simulink model "Prey_Predator_STM32F4"  (R2025a)
settings: Solver=FixedStepDiscrete  StartTime=0.0  StopTime=10.0  RelTol=1e-3
PreLoadFcn:
  | waijung.modelPreload; % Required for working with Waijung Blockset. Do not remove.
undefined symbols (not defined in the file): HSEOSC, Link, LQFP176, ST, STM32F417IG
libraries: stm32f4_io_lib x144, fuzblock x1, stm32f4_device_config_lib x1
(part 1 of 3)
CloseFcn:
  | waijung.modelClose; % Required for working with Waijung Blockset. Do not remove.
settings Model: Creator=Krisada  LastModifiedBy=prizy
settings SolverCC: AlgebraicLoopSolver=TrustRegion
settings DataIOCC: LimitDataPoints=on  SaveFormat=Array  SignalLoggingSaveFormat=ModelDataLogs  ReturnWorkspaceOutputs=off
settings OptimizationCC: ExpressionDepthLimit=2147483647.0  LifeSpan=1  EfficientTunableParamExpr=on
settings DebuggingCC: UnderspecifiedInitializationDetection=Classic  MergeDetectMultiDrivingBlocksExec=none  SolverPrmCheckMsg=warning  ParameterPrecisionLossMsg=none  FcnCallInpInsideContextMsg=warning  UnconnectedInputMsg=warning  UnconnectedOutputMsg=warning  UnconnectedLineMsg=warning  StateNameClashWarn=warning  SFUnexpectedBacktrackingDiag=warning  SFNoUnconditionalDefaultTransitionDiag=warning  SFExecutionAtInitializationDiag=none  ArithmeticOperatorsInVariantConditions=warning
settings HardwareCC: ProdBitPerPointer=32.0  ProdBitPerSizeT=32.0  ProdBitPerPtrDiffT=32.0  ProdLargestAtomicFloat=None  ProdIntDivRoundTo=Undefined  ProdWordSize=32.0  ProdHWDeviceType=ARM Compatible->Cortex - M4  TargetEndianess=LittleEndian  TargetHWDeviceType=ARM Compatible->Cortex - M4
settings ModelReferenceCC: PropagateSignalLabelsOutOfModel=off
settings SFSimCC: SimUseLocalCustomCode=off  MATLABDynamicMemAlloc=off  CustomCodeUndefinedFunction=UseInterfaceOnly
settings RTWCC: SystemTargetFile=stm32f4.tlc  GenerateMakefile=off  TemplateMakefile=ert_default_tmf  RTWUseLocalCustomCode=off  GPUComputeCapability=3.5  Description=STM32F4 Target
settings CodeAppCC: IgnoreCustomStorageClasses=off  CustomSymbolStrType=$N$R$M  StateflowObjectComments=on  InternalIdentifier=Classic
settings STFCustomTargetCC: SystemTargetFile=stm32f4.tlc  MultiwordLength=2048.0  DynamicStringBufferSize=256.0  ModelReferenceCompliant=off  CombineOutputUpdateFcns=on  ERTCustomFileBanners=on  SupportContinuousTime=off  SupportNonInlinedSFcns=off  RemoveResetFunc=on  MATLABClassNameForMDSCustomization=Simulink.SoftwareTarget.ERTCustomization  GRTInterface=off
settings ERTTargetCC: ExtModeTransport=0.0  ExtModeStaticAlloc=off  ExtModeMexFile=noextcomm  ExtModeIntrfLevel=Level1  InlinedParameterPlacement=Hierarchical  ERTSrcFileBannerTemplate=stm32f4_code_template.cgt  ERTHdrFileBannerTemplate=stm32f4_code_template.cgt  ERTDataSrcFileTemplate=stm32f4_code_template.cgt  ERTDataHdrFileTemplate=stm32f4_code_template.cgt  ERTCustomFileTemplate=stm32f4_file_process.tlc  ConvertIfToSwitch=off  SuppressUnreachableDefaultCases=off  DynamicArrayContainerType=coder::array  MultiwordLength=2048.0  ModelReferenceCompliant=off  ParMdlRefBuildCompliant=off  CompOptLevelCompliant=off  ConcurrentExecutionCompliant=off  ModelStepFunctionPrototypeControlCompliant=off  CPPClassGenCompliant=off  UseToolchainInfoCompliant=off
settings ConfigComp: CovMetricSettings=dw  CovSaveCumulativeToWorkspaceVar=on  CovSaveSingleToWorkspaceVar=on  CovExternalEMLEnable=off

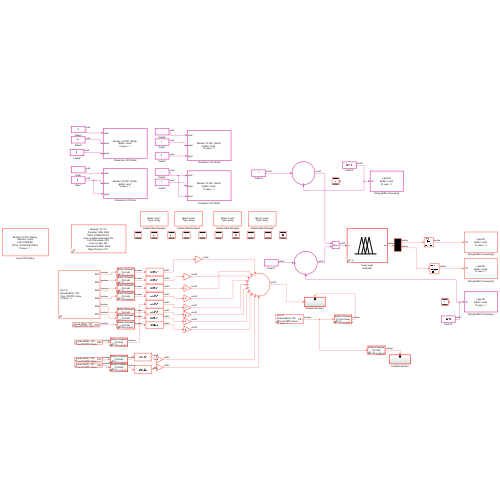
[thumbnail: Simulink's stored preview of the top-level diagram]
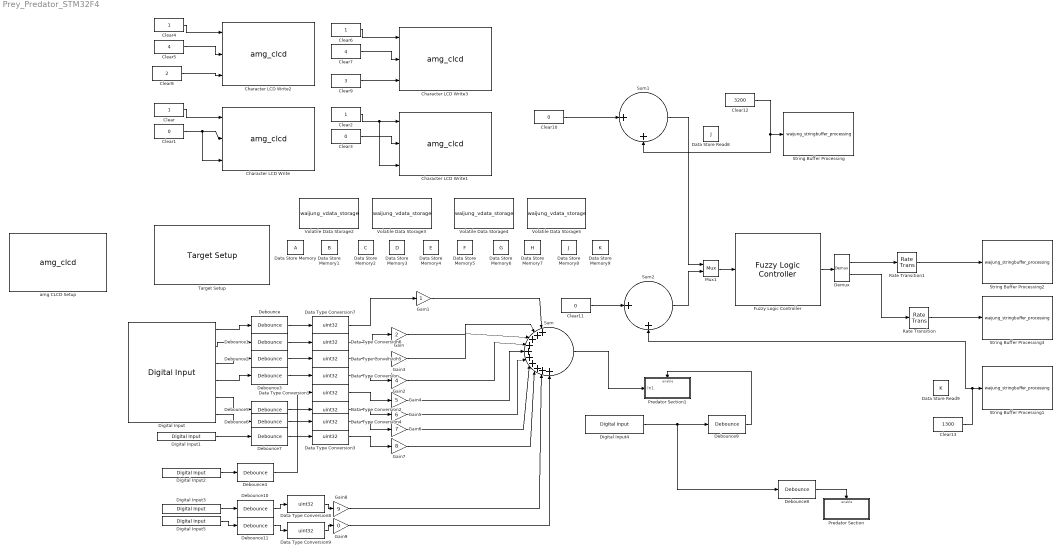
== system Prey_Predator_STM32F4 ==
  Character LCD Write : S-Function  FunctionName=amg_clcd  Parameters=module,configuration,inputtypearray,outputtypearray,confstr,sampletime,sampletimestr,blockid  SFunctionDeploymentMode=off  EnableBusSupport=off  mask(amg_clcd){configuration=Transaction, module=1, model=amg CLCD Std, interface=4-bits, linecount=4, columncount=20, gpiotype=Push-pull, controlport=E, control_rs=15, control_rw=13, control_en=11, dataport=A, data0=7, data1=5, data2=3, data3=1, usestringbuffer=on, stringbuffer=Line1, varname=VolatileDataStorage2_Line1, inputtypearray=[3 -1 -1 -1], outputtypearray=[0], confstr=["4","4","20","PP","E","15","11","13","","A","","","","","7","5","3","1","1","VolatileDataStorage2_Line1","1","0","0","0","1","0","0","0","0","stm32f4"], sampletime=-1, sampletimestr=-1, blockid=CharacterLCDWrite}
      mask prompts: model "LCD model:"; linecount "Number of lines:"; columncount "Number of columns:"; gpiotype "GPIO Output type:"; controlport "GPIO control port:"; control_rs "GPIO control pin, RS:"; control_rw "GPIO control pin, RW:"; control_en "GPIO control pin, EN:"; dataport "GPIO data D[7:4] port"; data0 "GPIO data pin, D4:"; data1 "GPIO data pin, D5:"; data2 "GPIO data pin, D6:"; data3 "GPIO data pin, D7:"; usestringbuffer "Use string buffer"; stringbuffer "String buffer"; varname "Variable name"; inputtypearray "Input type array"; outputtypearray "Output type array"; confstr "Configuration string"; sampletime "Sample time (sec)"; sampletimestr "Compiled sample time (sec) in string"
      mask help:
      | Note for cmd:
      | 1 - Clear specified LCD line display before write data to LCD.
      | Otherwise (e.g. 0) - Write data without clearing LCD Line.
      |
      | Position:
      | x = 0, First Character (from left to right)
      | y = 0, Top Line
      mask init:
      | amg_clcd_callback('init');
      mask Help: web(fullfile(waijungdocroot,'amg_clcd_write.htm'), '-browser')
      mask TypeOptions configuration: Setup | Transaction
      mask Callback configuration: amg_clcd_callback('configuration');
      mask TypeOptions module: 1 | 2 | 3 | 4
      mask TypeOptions model: amg CLCD Std
      mask TypeOptions interface: 4-bits
      mask TypeOptions gpiotype: Push-pull | Open-drain
      mask TypeOptions controlport: A | B | C | D | E | F | G | H | I
      mask TypeOptions control_rs: 0 | 1 | 2 | 3 | 4 | 5 | 6 | 7 | 8 | 9 | 10 | 11 | 12 | 13 | 14 | 15
      mask TypeOptions control_rw: 0 | 1 | 2 | 3 | 4 | 5 | 6 | 7 | 8 | 9 | 10 | 11 | 12 | 13 | 14 | 15
      mask TypeOptions control_en: 0 | 1 | 2 | 3 | 4 | 5 | 6 | 7 | 8 | 9 | 10 | 11 | 12 | 13 | 14 | 15
      mask TypeOptions dataport: A | B | C | D | E | F | G | H | I
      mask TypeOptions data0: 0 | 1 | 2 | 3 | 4 | 5 | 6 | 7 | 8 | 9 | 10 | 11 | 12 | 13 | 14 | 15
      mask TypeOptions data1: 0 | 1 | 2 | 3 | 4 | 5 | 6 | 7 | 8 | 9 | 10 | 11 | 12 | 13 | 14 | 15
      mask TypeOptions data2: 0 | 1 | 2 | 3 | 4 | 5 | 6 | 7 | 8 | 9 | 10 | 11 | 12 | 13 | 14 | 15
      mask TypeOptions data3: 0 | 1 | 2 | 3 | 4 | 5 | 6 | 7 | 8 | 9 | 10 | 11 | 12 | 13 | 14 | 15
      mask Callback usestringbuffer: amg_clcd_callback('usestringbuffer');
      mask TypeOptions stringbuffer: Line1 | Line2 | Line3 | Line4
      mask Callback varname: amg_clcd_callback('varname');
      mask Callback confstr: amg_clcd_callback('confstr');
      mask Callback sampletime: amg_clcd_callback('sampletime');
      mask Callback sampletimestr: amg_clcd_callback('sampletimestr');
      mask Callback blockid: amg_clcd_callback('blockid');
      mask Display: text(0.5, 0.5, 'Module: CLCD1 (Write)\nBuffer: Line1\nTs (sec): -1','ver','middle','hor','center');port_label('input', 1,'cmd');port_label('input', 2,'xpos');port_label('input', 3,'ypos');
  Character LCD Write1 : S-Function  FunctionName=amg_clcd  Parameters=module,configuration,inputtypearray,outputtypearray,confstr,sampletime,sampletimestr,blockid  SFunctionDeploymentMode=off  EnableBusSupport=off  mask(amg_clcd){configuration=Transaction, module=1, model=amg CLCD Std, interface=4-bits, linecount=4, columncount=20, gpiotype=Push-pull, controlport=E, control_rs=15, control_rw=13, control_en=11, dataport=A, data0=7, data1=5, data2=3, data3=1, usestringbuffer=on, stringbuffer=Line2, varname=VolatileDataStorage3_Line2, inputtypearray=[3 -1 -1 -1], outputtypearray=[0], confstr=["4","4","20","PP","E","15","11","13","","A","","","","","7","5","3","1","1","VolatileDataStorage3_Line2","1","0","0","0","1","0","0","0","0","stm32f4"], sampletime=-1, sampletimestr=-1, blockid=CharacterLCDWrite1}
      mask prompts: model "LCD model:"; linecount "Number of lines:"; columncount "Number of columns:"; gpiotype "GPIO Output type:"; controlport "GPIO control port:"; control_rs "GPIO control pin, RS:"; control_rw "GPIO control pin, RW:"; control_en "GPIO control pin, EN:"; dataport "GPIO data D[7:4] port"; data0 "GPIO data pin, D4:"; data1 "GPIO data pin, D5:"; data2 "GPIO data pin, D6:"; data3 "GPIO data pin, D7:"; usestringbuffer "Use string buffer"; stringbuffer "String buffer"; varname "Variable name"; inputtypearray "Input type array"; outputtypearray "Output type array"; confstr "Configuration string"; sampletime "Sample time (sec)"; sampletimestr "Compiled sample time (sec) in string"
      mask help:
      | Note for cmd:
      | 1 - Clear specified LCD line display before write data to LCD.
      | Otherwise (e.g. 0) - Write data without clearing LCD Line.
      |
      | Position:
      | x = 0, First Character (from left to right)
      | y = 0, Top Line
      mask init:
      | amg_clcd_callback('init');
      mask Help: web(fullfile(waijungdocroot,'amg_clcd_write.htm'), '-browser')
      mask TypeOptions configuration: Setup | Transaction
      mask Callback configuration: amg_clcd_callback('configuration');
      mask TypeOptions module: 1 | 2 | 3 | 4
      mask TypeOptions model: amg CLCD Std
      mask TypeOptions interface: 4-bits
      mask TypeOptions gpiotype: Push-pull | Open-drain
      mask TypeOptions controlport: A | B | C | D | E | F | G | H | I
      mask TypeOptions control_rs: 0 | 1 | 2 | 3 | 4 | 5 | 6 | 7 | 8 | 9 | 10 | 11 | 12 | 13 | 14 | 15
      mask TypeOptions control_rw: 0 | 1 | 2 | 3 | 4 | 5 | 6 | 7 | 8 | 9 | 10 | 11 | 12 | 13 | 14 | 15
      mask TypeOptions control_en: 0 | 1 | 2 | 3 | 4 | 5 | 6 | 7 | 8 | 9 | 10 | 11 | 12 | 13 | 14 | 15
      mask TypeOptions dataport: A | B | C | D | E | F | G | H | I
      mask TypeOptions data0: 0 | 1 | 2 | 3 | 4 | 5 | 6 | 7 | 8 | 9 | 10 | 11 | 12 | 13 | 14 | 15
      mask TypeOptions data1: 0 | 1 | 2 | 3 | 4 | 5 | 6 | 7 | 8 | 9 | 10 | 11 | 12 | 13 | 14 | 15
      mask TypeOptions data2: 0 | 1 | 2 | 3 | 4 | 5 | 6 | 7 | 8 | 9 | 10 | 11 | 12 | 13 | 14 | 15
      mask TypeOptions data3: 0 | 1 | 2 | 3 | 4 | 5 | 6 | 7 | 8 | 9 | 10 | 11 | 12 | 13 | 14 | 15
      mask Callback usestringbuffer: amg_clcd_callback('usestringbuffer');
      mask TypeOptions stringbuffer: Line1 | Line2 | Line3 | Line4
      mask Callback varname: amg_clcd_callback('varname');
      mask Callback confstr: amg_clcd_callback('confstr');
      mask Callback sampletime: amg_clcd_callback('sampletime');
      mask Callback sampletimestr: amg_clcd_callback('sampletimestr');
      mask Callback blockid: amg_clcd_callback('blockid');
      mask Display: text(0.5, 0.5, 'Module: CLCD1 (Write)\nBuffer: Line2\nTs (sec): -1','ver','middle','hor','center');port_label('input', 1,'cmd');port_label('input', 2,'xpos');port_label('input', 3,'ypos');
  Character LCD Write2 : S-Function  FunctionName=amg_clcd  Parameters=module,configuration,inputtypearray,outputtypearray,confstr,sampletime,sampletimestr,blockid  SFunctionDeploymentMode=off  EnableBusSupport=off  mask(amg_clcd){configuration=Transaction, module=1, model=amg CLCD Std, interface=4-bits, linecount=4, columncount=20, gpiotype=Push-pull, controlport=E, control_rs=15, control_rw=13, control_en=11, dataport=A, data0=7, data1=5, data2=3, data3=1, usestringbuffer=on, stringbuffer=Line3, varname=VolatileDataStorage4_Line3, inputtypearray=[3 -1 -1 -1], outputtypearray=[0], confstr=["4","4","20","PP","E","15","11","13","","A","","","","","7","5","3","1","1","VolatileDataStorage4_Line3","1","0","0","0","1","0","0","0","0","stm32f4"], sampletime=-1, sampletimestr=-1, blockid=CharacterLCDWrite2}
      mask prompts: model "LCD model:"; linecount "Number of lines:"; columncount "Number of columns:"; gpiotype "GPIO Output type:"; controlport "GPIO control port:"; control_rs "GPIO control pin, RS:"; control_rw "GPIO control pin, RW:"; control_en "GPIO control pin, EN:"; dataport "GPIO data D[7:4] port"; data0 "GPIO data pin, D4:"; data1 "GPIO data pin, D5:"; data2 "GPIO data pin, D6:"; data3 "GPIO data pin, D7:"; usestringbuffer "Use string buffer"; stringbuffer "String buffer"; varname "Variable name"; inputtypearray "Input type array"; outputtypearray "Output type array"; confstr "Configuration string"; sampletime "Sample time (sec)"; sampletimestr "Compiled sample time (sec) in string"
      mask help:
      | Note for cmd:
      | 1 - Clear specified LCD line display before write data to LCD.
      | Otherwise (e.g. 0) - Write data without clearing LCD Line.
      |
      | Position:
      | x = 0, First Character (from left to right)
      | y = 0, Top Line
      mask init:
      | amg_clcd_callback('init');
      mask Help: web(fullfile(waijungdocroot,'amg_clcd_write.htm'), '-browser')
      mask TypeOptions configuration: Setup | Transaction
      mask Callback configuration: amg_clcd_callback('configuration');
      mask TypeOptions module: 1 | 2 | 3 | 4
      mask TypeOptions model: amg CLCD Std
      mask TypeOptions interface: 4-bits
      mask TypeOptions gpiotype: Push-pull | Open-drain
      mask TypeOptions controlport: A | B | C | D | E | F | G | H | I
      mask TypeOptions control_rs: 0 | 1 | 2 | 3 | 4 | 5 | 6 | 7 | 8 | 9 | 10 | 11 | 12 | 13 | 14 | 15
      mask TypeOptions control_rw: 0 | 1 | 2 | 3 | 4 | 5 | 6 | 7 | 8 | 9 | 10 | 11 | 12 | 13 | 14 | 15
      mask TypeOptions control_en: 0 | 1 | 2 | 3 | 4 | 5 | 6 | 7 | 8 | 9 | 10 | 11 | 12 | 13 | 14 | 15
      mask TypeOptions dataport: A | B | C | D | E | F | G | H | I
      mask TypeOptions data0: 0 | 1 | 2 | 3 | 4 | 5 | 6 | 7 | 8 | 9 | 10 | 11 | 12 | 13 | 14 | 15
      mask TypeOptions data1: 0 | 1 | 2 | 3 | 4 | 5 | 6 | 7 | 8 | 9 | 10 | 11 | 12 | 13 | 14 | 15
      mask TypeOptions data2: 0 | 1 | 2 | 3 | 4 | 5 | 6 | 7 | 8 | 9 | 10 | 11 | 12 | 13 | 14 | 15
      mask TypeOptions data3: 0 | 1 | 2 | 3 | 4 | 5 | 6 | 7 | 8 | 9 | 10 | 11 | 12 | 13 | 14 | 15
      mask Callback usestringbuffer: amg_clcd_callback('usestringbuffer');
      mask TypeOptions stringbuffer: Line1 | Line2 | Line3 | Line4
      mask Callback varname: amg_clcd_callback('varname');
      mask Callback confstr: amg_clcd_callback('confstr');
      mask Callback sampletime: amg_clcd_callback('sampletime');
      mask Callback sampletimestr: amg_clcd_callback('sampletimestr');
      mask Callback blockid: amg_clcd_callback('blockid');
      mask Display: text(0.5, 0.5, 'Module: CLCD1 (Write)\nBuffer: Line3\nTs (sec): -1','ver','middle','hor','center');port_label('input', 1,'cmd');port_label('input', 2,'xpos');port_label('input', 3,'ypos');
  Character LCD Write3 : S-Function  FunctionName=amg_clcd  Parameters=module,configuration,inputtypearray,outputtypearray,confstr,sampletime,sampletimestr,blockid  SFunctionDeploymentMode=off  EnableBusSupport=off  mask(amg_clcd){configuration=Transaction, module=1, model=amg CLCD Std, interface=4-bits, linecount=4, columncount=20, gpiotype=Push-pull, controlport=E, control_rs=15, control_rw=13, control_en=11, dataport=A, data0=7, data1=5, data2=3, data3=1, usestringbuffer=on, stringbuffer=Line4, varname=VolatileDataStorage5_Line4, inputtypearray=[3 -1 -1 -1], outputtypearray=[0], confstr=["4","4","20","PP","E","15","11","13","","A","","","","","7","5","3","1","1","VolatileDataStorage5_Line4","1","0","0","0","1","0","0","0","0","stm32f4"], sampletime=-1, sampletimestr=-1, blockid=CharacterLCDWrite3}
      mask prompts: model "LCD model:"; linecount "Number of lines:"; columncount "Number of columns:"; gpiotype "GPIO Output type:"; controlport "GPIO control port:"; control_rs "GPIO control pin, RS:"; control_rw "GPIO control pin, RW:"; control_en "GPIO control pin, EN:"; dataport "GPIO data D[7:4] port"; data0 "GPIO data pin, D4:"; data1 "GPIO data pin, D5:"; data2 "GPIO data pin, D6:"; data3 "GPIO data pin, D7:"; usestringbuffer "Use string buffer"; stringbuffer "String buffer"; varname "Variable name"; inputtypearray "Input type array"; outputtypearray "Output type array"; confstr "Configuration string"; sampletime "Sample time (sec)"; sampletimestr "Compiled sample time (sec) in string"
      mask help:
      | Note for cmd:
      | 1 - Clear specified LCD line display before write data to LCD.
      | Otherwise (e.g. 0) - Write data without clearing LCD Line.
      |
      | Position:
      | x = 0, First Character (from left to right)
      | y = 0, Top Line
      mask init:
      | amg_clcd_callback('init');
      mask Help: web(fullfile(waijungdocroot,'amg_clcd_write.htm'), '-browser')
      mask TypeOptions configuration: Setup | Transaction
      mask Callback configuration: amg_clcd_callback('configuration');
      mask TypeOptions module: 1 | 2 | 3 | 4
      mask TypeOptions model: amg CLCD Std
      mask TypeOptions interface: 4-bits
      mask TypeOptions gpiotype: Push-pull | Open-drain
      mask TypeOptions controlport: A | B | C | D | E | F | G | H | I
      mask TypeOptions control_rs: 0 | 1 | 2 | 3 | 4 | 5 | 6 | 7 | 8 | 9 | 10 | 11 | 12 | 13 | 14 | 15
      mask TypeOptions control_rw: 0 | 1 | 2 | 3 | 4 | 5 | 6 | 7 | 8 | 9 | 10 | 11 | 12 | 13 | 14 | 15
      mask TypeOptions control_en: 0 | 1 | 2 | 3 | 4 | 5 | 6 | 7 | 8 | 9 | 10 | 11 | 12 | 13 | 14 | 15
      mask TypeOptions dataport: A | B | C | D | E | F | G | H | I
      mask TypeOptions data0: 0 | 1 | 2 | 3 | 4 | 5 | 6 | 7 | 8 | 9 | 10 | 11 | 12 | 13 | 14 | 15
      mask TypeOptions data1: 0 | 1 | 2 | 3 | 4 | 5 | 6 | 7 | 8 | 9 | 10 | 11 | 12 | 13 | 14 | 15
      mask TypeOptions data2: 0 | 1 | 2 | 3 | 4 | 5 | 6 | 7 | 8 | 9 | 10 | 11 | 12 | 13 | 14 | 15
      mask TypeOptions data3: 0 | 1 | 2 | 3 | 4 | 5 | 6 | 7 | 8 | 9 | 10 | 11 | 12 | 13 | 14 | 15
      mask Callback usestringbuffer: amg_clcd_callback('usestringbuffer');
      mask TypeOptions stringbuffer: Line1 | Line2 | Line3 | Line4
      mask Callback varname: amg_clcd_callback('varname');
      mask Callback confstr: amg_clcd_callback('confstr');
      mask Callback sampletime: amg_clcd_callback('sampletime');
      mask Callback sampletimestr: amg_clcd_callback('sampletimestr');
      mask Callback blockid: amg_clcd_callback('blockid');
      mask Display: text(0.5, 0.5, 'Module: CLCD1 (Write)\nBuffer: Line4\nTs (sec): -1','ver','middle','hor','center');port_label('input', 1,'cmd');port_label('input', 2,'xpos');port_label('input', 3,'ypos');
  Clear{,2,4,6} (4 alike) : Constant  OutDataTypeStr=uint8
  Clear1 : Constant  Value=0  OutDataTypeStr=uint8
  Clear10 : Constant  Value=0  OutDataTypeStr=uint32
  Clear11 : Constant  Value=0  OutDataTypeStr=uint32
  Clear12 : Constant  Value=3200  OutDataTypeStr=uint32
  Clear13 : Constant  Value=1300  OutDataTypeStr=uint32
  Clear3 : Constant  Value=0  OutDataTypeStr=uint8
  Clear5 : Constant  Value=4  OutDataTypeStr=uint8
  Clear7 : Constant  Value=4  OutDataTypeStr=uint8
  Clear8 : Constant  Value=2  OutDataTypeStr=uint8
  Clear9 : Constant  Value=3  OutDataTypeStr=uint8
  Data Store Memory : DataStoreMemory  ReadBeforeWriteMsg=warning  WriteAfterWriteMsg=warning  WriteAfterReadMsg=warning  ShowAdditionalParam=off
  Data Store Memory1 : DataStoreMemory  DataStoreName=B  ReadBeforeWriteMsg=warning  WriteAfterWriteMsg=warning  WriteAfterReadMsg=warning  ShowAdditionalParam=off
  Data Store Memory2 : DataStoreMemory  DataStoreName=C  ReadBeforeWriteMsg=warning  WriteAfterWriteMsg=warning  WriteAfterReadMsg=warning  ShowAdditionalParam=off
  Data Store Memory3 : DataStoreMemory  DataStoreName=D  ReadBeforeWriteMsg=warning  WriteAfterWriteMsg=warning  WriteAfterReadMsg=warning  ShowAdditionalParam=off
  Data Store Memory4 : DataStoreMemory  DataStoreName=E  ReadBeforeWriteMsg=warning  WriteAfterWriteMsg=warning  WriteAfterReadMsg=warning  ShowAdditionalParam=off
  Data Store Memory5 : DataStoreMemory  DataStoreName=F  ReadBeforeWriteMsg=warning  WriteAfterWriteMsg=warning  WriteAfterReadMsg=warning  ShowAdditionalParam=off
  Data Store Memory6 : DataStoreMemory  DataStoreName=G  ReadBeforeWriteMsg=warning  WriteAfterWriteMsg=warning  WriteAfterReadMsg=warning  ShowAdditionalParam=off
  Data Store Memory7 : DataStoreMemory  DataStoreName=H  ReadBeforeWriteMsg=warning  WriteAfterWriteMsg=warning  WriteAfterReadMsg=warning  ShowAdditionalParam=off
  Data Store Memory8 : DataStoreMemory  DataStoreName=J  ReadBeforeWriteMsg=warning  WriteAfterWriteMsg=warning  WriteAfterReadMsg=warning  ShowAdditionalParam=off
  Data Store Memory9 : DataStoreMemory  DataStoreName=K  ReadBeforeWriteMsg=warning  WriteAfterWriteMsg=warning  WriteAfterReadMsg=warning  ShowAdditionalParam=off
  Data Store Read8 : DataStoreRead  DataStoreName=J  IndexOptions=Index vector (dialog)  Indices=1  OutputSizes=1
  Data Store Read9 : DataStoreRead  DataStoreName=K  IndexOptions=Index vector (dialog)  Indices=1  OutputSizes=1
  Data Type Conversion{,1..9} (10 alike) : DataTypeConversion  OutDataTypeStr=uint32  SaturateOnIntegerOverflow=off  RndMeth=Floor
  Debounce{,1..8,10..11} (11 alike) : stm32f4_io_lib/Debounce  mode=Normal  prescale=4  debounce=4
      settings: SourceProductName=IO
  Debounce9 : stm32f4_io_lib/Debounce  mode=Single Pulse  prescale=4  debounce=4
      settings: SourceProductName=IO
  Demux : Demux  Outputs=2
  Digital Input : stm32f4_io_lib/Digital Input  port=D  speed=100  porttype=None  porttypestr=NOPULL  use_pin0=off  use_pin1=on  use_pin2=on  use_pin3=on  use_pin4=on  use_pin5=off  use_pin6=on  use_pin7=on  use_pin8=off  use_pin9=off  use_pin10=off  use_pin11=off  use_pin12=off  use_pin13=off  use_pin14=off  use_pin15=off  pinstr=GPIO_Pin_1 | GPIO_Pin_2 | GPIO_Pin_3 | GPIO_Pin_4 | GPIO_Pin_6 | GPIO_Pin_7  usedpinarray="[0  1  1  1  1  0  1  1  0  0  0  0  0  0  0  0]"  bitbandingstr=|  sampletime=0.01  sampletimestr=-1  blockid=DigitalInput  enablecustomportlabel=off  glabalinit=off  cinputportlabel=In1, In2  coutputportlabel=Out1, Out2
      | #define DigitalInput_D1 Peripheral_BB(GPIOD->IDR, 1)  /* Output pin */
      | #define DigitalInput_D2 Peripheral_BB(GPIOD->IDR, 2)  /* Output pin */
      | #define DigitalInput_D3 Peripheral_BB(GPIOD->IDR, 3)  /* Output pin */
      | #define DigitalInput_D4 Peripheral_BB(GPIOD->IDR, 4)  /* Output pin */
      | #define DigitalInput_D6 Peripheral_BB(GPIOD->IDR, 6)  /* Output pin */
      | #define DigitalInput_D7 Peripheral_BB(GPIOD->IDR, 7)  /* Output pin */
      settings: SourceProductName=IO
  Digital Input1 : stm32f4_io_lib/Digital Input  port=B  speed=100  porttype=None  porttypestr=NOPULL  use_pin0=off  use_pin1=off  use_pin2=off  use_pin3=on  use_pin4=off  use_pin5=off  use_pin6=off  use_pin7=off  use_pin8=off  use_pin9=off  use_pin10=off  use_pin11=off  use_pin12=off  use_pin13=off  use_pin14=off  use_pin15=off  pinstr=GPIO_Pin_3  usedpinarray="[0  0  0  1  0  0  0  0  0  0  0  0  0  0  0  0]"  bitbandingstr="#define DigitalInput1_B3 Peripheral_BB(GPIOB->IDR, 3)  /* Output pin */"  sampletime=0.01  sampletimestr=-1  blockid=DigitalInput1  enablecustomportlabel=off  glabalinit=off  cinputportlabel=In1, In2  coutputportlabel=Out1, Out2
      settings: SourceProductName=IO
  Digital Input2 : stm32f4_io_lib/Digital Input  port=B  speed=100  porttype=None  porttypestr=NOPULL  use_pin0=off  use_pin1=off  use_pin2=off  use_pin3=off  use_pin4=off  use_pin5=on  use_pin6=off  use_pin7=off  use_pin8=off  use_pin9=off  use_pin10=off  use_pin11=off  use_pin12=off  use_pin13=off  use_pin14=off  use_pin15=off  pinstr=GPIO_Pin_5  usedpinarray="[0  0  0  0  0  1  0  0  0  0  0  0  0  0  0  0]"  bitbandingstr="#define DigitalInput2_B5 Peripheral_BB(GPIOB->IDR, 5)  /* Output pin */"  sampletime=0.01  sampletimestr=-1  blockid=DigitalInput2  enablecustomportlabel=off  glabalinit=off  cinputportlabel=In1, In2  coutputportlabel=Out1, Out2
      settings: SourceProductName=IO
  Digital Input3 : stm32f4_io_lib/Digital Input  port=A  speed=100  porttype=None  porttypestr=NOPULL  use_pin0=off  use_pin1=on  use_pin2=off  use_pin3=off  use_pin4=off  use_pin5=off  use_pin6=off  use_pin7=off  use_pin8=off  use_pin9=off  use_pin10=off  use_pin11=off  use_pin12=off  use_pin13=off  use_pin14=off  use_pin15=off  pinstr=GPIO_Pin_1  usedpinarray="[0  1  0  0  0  0  0  0  0  0  0  0  0  0  0  0]"  bitbandingstr="#define DigitalInput3_A1 Peripheral_BB(GPIOA->IDR, 1)  /* Output pin */"  sampletime=0.01  sampletimestr=-1  blockid=DigitalInput3  enablecustomportlabel=off  glabalinit=off  cinputportlabel=In1, In2  coutputportlabel=Out1, Out2
      settings: SourceProductName=IO
  Digital Input4 : stm32f4_io_lib/Digital Input  port=E  speed=100  porttype=None  porttypestr=NOPULL  use_pin0=off  use_pin1=on  use_pin2=off  use_pin3=off  use_pin4=off  use_pin5=off  use_pin6=off  use_pin7=off  use_pin8=off  use_pin9=off  use_pin10=off  use_pin11=off  use_pin12=off  use_pin13=off  use_pin14=off  use_pin15=off  pinstr=GPIO_Pin_1  usedpinarray="[0  1  0  0  0  0  0  0  0  0  0  0  0  0  0  0]"  bitbandingstr="#define DigitalInput4_E1 Peripheral_BB(GPIOE->IDR, 1)  /* Output pin */"  sampletime=0.01  sampletimestr=-1  blockid=DigitalInput4  enablecustomportlabel=off  glabalinit=off  cinputportlabel=In1, In2  coutputportlabel=Out1, Out2
      settings: SourceProductName=IO
  Digital Input5 : stm32f4_io_lib/Digital Input  port=A  speed=100  porttype=None  porttypestr=NOPULL  use_pin0=on  use_pin1=off  use_pin2=off  use_pin3=off  use_pin4=off  use_pin5=off  use_pin6=off  use_pin7=off  use_pin8=off  use_pin9=off  use_pin10=off  use_pin11=off  use_pin12=off  use_pin13=off  use_pin14=off  use_pin15=off  pinstr=GPIO_Pin_0  usedpinarray="[1  0  0  0  0  0  0  0  0  0  0  0  0  0  0  0]"  bitbandingstr="#define DigitalInput5_A0 Peripheral_BB(GPIOA->IDR, 0)  /* Output pin */"  sampletime=0.01  sampletimestr=-1  blockid=DigitalInput5  enablecustomportlabel=off  glabalinit=off  cinputportlabel=In1, In2  coutputportlabel=Out1, Out2
      settings: SourceProductName=IO
  Fuzzy Logic Controller : fuzblock/Fuzzy Logic  Controller  FIS=fismat  OutputSampleNumber=101  DataType=double  UseLookupTable=off  NumBreakpoints=10  FuzzifiedInputs=off  RuleFiringStrengths=off  RuleOutputs=off  AggregatedOutputs=off  SimulateUsing=Interpreted execution  OutOfRangeInputValueMessage=warning  NoRuleFiredMessage=warning  EmptyOutputFuzzySetMessage=warning
  Gain : Gain  Gain=2  OutDataTypeStr=Inherit: Same as input
  Gain1 : Gain  OutDataTypeStr=Inherit: Same as input
  Gain2 : Gain  Gain=4  OutDataTypeStr=Inherit: Same as input
  Gain3 : Gain  Gain=3  OutDataTypeStr=Inherit: Same as input
  Gain4 : Gain  Gain=5  OutDataTypeStr=Inherit: Same as input
  Gain5 : Gain  Gain=6  OutDataTypeStr=Inherit: Same as input
  Gain6 : Gain  Gain=7  OutDataTypeStr=Inherit: Same as input
  Gain7 : Gain  Gain=8  OutDataTypeStr=Inherit: Same as input
  Gain8 : Gain  Gain=9  OutDataTypeStr=Inherit: Same as input
  Gain9 : Gain  Gain=0  OutDataTypeStr=Inherit: Same as input
  Mux1 : Mux  Inputs=2
  Predator Section : Subsystem
  Predator Section1 : Subsystem
  Rate Transition : RateTransition  OutPortSampleTimeOpt=Inherit
  Rate Transition1 : RateTransition  OutPortSampleTimeOpt=Inherit
  String Buffer Processing : S-Function  FunctionName=waijung_stringbuffer_processing  Parameters=configuration,varname,sformat,porttypes,portcount,inputtypearray,outputtypearray,sampletime,sampletimestr,blockid  SFunctionDeploymentMode=off  EnableBusSupport=off  mask(waijung_stringbuffer_processing){configuration=sprintf, storagename=Line3, sformat='Prey: %1.0f', enableoutput=off, varname=VolatileDataStorage4_Line3, inputtypearray=[1 -1], outputtypearray=[0], porttypes=["float"], portcount=1, sampletime=-1, sampletimestr=-1, blockid=StringBufferProcessing}
      mask prompts: configuration "Function"; storagename "String buffer"; sformat "Printf format"; enableoutput "Enable output status"; varname "Variable name"; inputtypearray "Input type array"; outputtypearray "Output type array"; porttypes "Port type list"; portcount "Port type count"; sampletime "Sample time (sec)"; sampletimestr "Compiled sample time (sec) in string"
      mask help:
      | This block implements string processing, sprintf/ sscanf command.
      | Supported format:
      | %u, %i, %o, %x: uint32
      | %d: int32
      | %e, %g, %f: single
      | %c: int8
      |
      | Status:
      |  0: Failed.
      |  Non-zero: Success.
      mask init:
      | waijung_stringbuffer_processing_callback('init');
      mask Help: web(fullfile(waijungdocroot,'String_Buffer_Processing.htm'))
      mask TypeOptions configuration: sprintf | sscanf
      mask Callback configuration: waijung_stringbuffer_processing_callback('configuration');
      mask TypeOptions storagename: Line1 | Line2 | Line3 | Line4 | <output>
      mask Callback sformat: waijung_stringbuffer_processing_callback('sformat');
      mask Callback enableoutput: waijung_stringbuffer_processing_callback('enableoutput');
      mask Callback sampletime: waijung_stringbuffer_processing_callback('sampletime');
      mask Callback sampletimestr: waijung_stringbuffer_processing_callback('sampletimestr');
      mask Callback blockid: waijung_stringbuffer_processing_callback('blockid');
      mask Display: text(0.5, 0.5, '[ sprintf ]\nBuffer: Line3\nTs (sec): -1','ver','middle','hor','center');port_label('input', 1,'%f');
  String Buffer Processing1 : S-Function  FunctionName=waijung_stringbuffer_processing  Parameters=configuration,varname,sformat,porttypes,portcount,inputtypearray,outputtypearray,sampletime,sampletimestr,blockid  SFunctionDeploymentMode=off  EnableBusSupport=off  mask(waijung_stringbuffer_processing){configuration=sprintf, storagename=Line4, sformat='Predator: %1.0f', enableoutput=off, varname=VolatileDataStorage5_Line4, inputtypearray=[1 -1], outputtypearray=[0], porttypes=["float"], portcount=1, sampletime=-1, sampletimestr=-1, blockid=StringBufferProcessing1}
      mask prompts: configuration "Function"; storagename "String buffer"; sformat "Printf format"; enableoutput "Enable output status"; varname "Variable name"; inputtypearray "Input type array"; outputtypearray "Output type array"; porttypes "Port type list"; portcount "Port type count"; sampletime "Sample time (sec)"; sampletimestr "Compiled sample time (sec) in string"
      mask help:
      | This block implements string processing, sprintf/ sscanf command.
      | Supported format:
      | %u, %i, %o, %x: uint32
      | %d: int32
      | %e, %g, %f: single
      | %c: int8
      |
      | Status:
      |  0: Failed.
      |  Non-zero: Success.
      mask init:
      | waijung_stringbuffer_processing_callback('init');
      mask Help: web(fullfile(waijungdocroot,'String_Buffer_Processing.htm'))
      mask TypeOptions configuration: sprintf | sscanf
      mask Callback configuration: waijung_stringbuffer_processing_callback('configuration');
      mask TypeOptions storagename: Line1 | Line2 | Line3 | Line4 | <output>
      mask Callback sformat: waijung_stringbuffer_processing_callback('sformat');
      mask Callback enableoutput: waijung_stringbuffer_processing_callback('enableoutput');
      mask Callback sampletime: waijung_stringbuffer_processing_callback('sampletime');
      mask Callback sampletimestr: waijung_stringbuffer_processing_callback('sampletimestr');
      mask Callback blockid: waijung_stringbuffer_processing_callback('blockid');
      mask Display: text(0.5, 0.5, '[ sprintf ]\nBuffer: Line4\nTs (sec): -1','ver','middle','hor','center');port_label('input', 1,'%f');
  String Buffer Processing2 : S-Function  FunctionName=waijung_stringbuffer_processing  Parameters=configuration,varname,sformat,porttypes,portcount,inputtypearray,outputtypearray,sampletime,sampletimestr,blockid  SFunctionDeploymentMode=off  EnableBusSupport=off  mask(waijung_stringbuffer_processing){configuration=sprintf, storagename=Line1, sformat='Prey: %1.2f', enableoutput=off, varname=VolatileDataStorage2_Line1, inputtypearray=[1 -1], outputtypearray=[0], porttypes=["float"], portcount=1, sampletime=-1, sampletimestr=-1, blockid=StringBufferProcessing2}
      mask prompts: configuration "Function"; storagename "String buffer"; sformat "Printf format"; enableoutput "Enable output status"; varname "Variable name"; inputtypearray "Input type array"; outputtypearray "Output type array"; porttypes "Port type list"; portcount "Port type count"; sampletime "Sample time (sec)"; sampletimestr "Compiled sample time (sec) in string"
      mask help:
      | This block implements string processing, sprintf/ sscanf command.
      | Supported format:
      | %u, %i, %o, %x: uint32
      | %d: int32
      | %e, %g, %f: single
      | %c: int8
      |
      | Status:
      |  0: Failed.
      |  Non-zero: Success.
      mask init:
      | waijung_stringbuffer_processing_callback('init');
      mask Help: web(fullfile(waijungdocroot,'String_Buffer_Processing.htm'))
      mask TypeOptions configuration: sprintf | sscanf
      mask Callback configuration: waijung_stringbuffer_processing_callback('configuration');
      mask TypeOptions storagename: Line1 | Line2 | Line3 | Line4 | <output>
      mask Callback sformat: waijung_stringbuffer_processing_callback('sformat');
      mask Callback enableoutput: waijung_stringbuffer_processing_callback('enableoutput');
      mask Callback sampletime: waijung_stringbuffer_processing_callback('sampletime');
      mask Callback sampletimestr: waijung_stringbuffer_processing_callback('sampletimestr');
      mask Callback blockid: waijung_stringbuffer_processing_callback('blockid');
      mask Display: text(0.5, 0.5, '[ sprintf ]\nBuffer: Line1\nTs (sec): -1','ver','middle','hor','center');port_label('input', 1,'%f');
  String Buffer Processing3 : S-Function  FunctionName=waijung_stringbuffer_processing  Parameters=configuration,varname,sformat,porttypes,portcount,inputtypearray,outputtypearray,sampletime,sampletimestr,blockid  SFunctionDeploymentMode=off  EnableBusSupport=off  mask(waijung_stringbuffer_processing){configuration=sprintf, storagename=Line2, sformat='Pdtor %1.0f', enableoutput=off, varname=VolatileDataStorage3_Line2, inputtypearray=[1 -1], outputtypearray=[0], porttypes=["float"], portcount=1, sampletime=-1, sampletimestr=-1, blockid=StringBufferProcessing3}
      mask prompts: configuration "Function"; storagename "String buffer"; sformat "Printf format"; enableoutput "Enable output status"; varname "Variable name"; inputtypearray "Input type array"; outputtypearray "Output type array"; porttypes "Port type list"; portcount "Port type count"; sampletime "Sample time (sec)"; sampletimestr "Compiled sample time (sec) in string"
      mask help:
      | This block implements string processing, sprintf/ sscanf command.
      | Supported format:
      | %u, %i, %o, %x: uint32
      | %d: int32
      | %e, %g, %f: single
      | %c: int8
      |
      | Status:
      |  0: Failed.
      |  Non-zero: Success.
      mask init:
      | waijung_stringbuffer_processing_callback('init');
      mask Help: web(fullfile(waijungdocroot,'String_Buffer_Processing.htm'))
      mask TypeOptions configuration: sprintf | sscanf
      mask Callback configuration: waijung_stringbuffer_processing_callback('configuration');
      mask TypeOptions storagename: Line1 | Line2 | Line3 | Line4 | <output>
      mask Callback sformat: waijung_stringbuffer_processing_callback('sformat');
      mask Callback enableoutput: waijung_stringbuffer_processing_callback('enableoutput');
      mask Callback sampletime: waijung_stringbuffer_processing_callback('sampletime');
      mask Callback sampletimestr: waijung_stringbuffer_processing_callback('sampletimestr');
      mask Callback blockid: waijung_stringbuffer_processing_callback('blockid');
      mask Display: text(0.5, 0.5, '[ sprintf ]\nBuffer: Line2\nTs (sec): -1','ver','middle','hor','center');port_label('input', 1,'%f');
  Sum : Sum  Inputs=|++++++++++
  Sum1 : Sum  Inputs=|++
  Sum2 : Sum  Inputs=|++
  Target Setup : stm32f4_device_config_lib/Target Setup  Priority=100  compiler=GNU ARM  previous_compiler=GNU ARM  mcu=STM32F417IG (LQFP176)  mcustr=STM32F417IG  clockconfig=HSEOSC-8MHz  system_stm32f4xx_c_path=C:\Users\prizy\Downloads\waijung_18.11a\targets\stm32f4_target\stm32f4\utils\system_stm32f4xx_default\STM32F40_41xxx\hseosc8mhz  showmemoryconfiguration=off  stacksize=0x400  heapsize=0x200  enableautocompiledownload=on  fullchiperase=off  programmerinterface=ST-Link  editctrlstr=on  compilercontrolstr=$(patsubst %, -I%, .) -mcpu=cortex-m4 -mthumb -mthumb-interwork -mfloat-abi=hard -mfpu=fpv4-sp-d16 -ffast-math -Wall -Wextra -Ofast  assemblercontrolstr=$(patsubst %, -I%, .) -mcpu=cortex-m4 -mthumb -mthumb-interwork -mfloat-abi=hard -mfpu=fpv4-sp-d16 -ffast-math -Wall -Wextra -Ofast -Wa,-amhls=$(<:.s=.lst) -D__STACK_SIZE=$(STACK_SIZE) -D__HEAP_SIZE=$(HEAP_SIZE)  linkercontrolstr=-T$(LD_SCRIPT) -g -Wl,-Map=$(MAP),--cref,--no-warn-mismatch -mcpu=cortex-m4 -mthumb -mthumb-interwork -mfloat-abi=hard -mfpu=fpv4-sp-d16  runafterdownload=on  execprofile=None  profileruart=1  profilerbaud=115200  profilertxpin=D8  profilerinitstr=0.01,168000000,1680000,115200,0  manualsetsampletime=off  sampletime=0.01  blockid=TargetSetup  systickreloadvalue=1680000  hseval=8000000  lastprofileruart=1  hclk=168000000  flashorigin=0x8000000  flashlength=1024k  ramorigin=0x20000000  ramlength=128k  useextram=off
      settings: SourceProductName=Device Configuration
  Volatile Data Storage2 : S-Function  FunctionName=waijung_vdata_storage  Parameters=storagetype,storagename,initval,varname,buffersize,initvalstring,sampletime,sampletimestr,blockid,storagetypestr  SFunctionDeploymentMode=off  EnableBusSupport=off  mask(waijung_vdata_storage){storagetype=string, storagename=Line1, initval=0, varname=VolatileDataStorage2_Line1, buffersize=64, initvalstring='', webintegration=Disable, weboutputformat='%s', webcgicallback=(void*)0, laststoragetype=string, sampletime=-1, sampletimestr=-1, blockid=VolatileDataStorage2, storagetypestr=char}
      mask prompts: storagetype "Storage Type"; storagename "Storage Name (must be a valid variable name)"; initval "Initial value (Apply at Power on Reset only)"; varname "Variable name"; buffersize "Size (bytes)"; initvalstring "Initial value (Apply at Power on Reset only)"; webintegration "Web CGI varget/varset integration"; weboutputformat "Web CGI varget output format"; webcgicallback "Web CGI varset callback"; laststoragetype "Last selected Storage Type"; sampletime "Sample time (sec)"; sampletimestr "Compiled sample time (sec) in string"; storagetypestr "Type string"
      mask help:
      | This block implements a volatile Data Storage.
      |
      | Web CGI varset/varget integratiopn:
      | Enable - In webserver application, allow remote access via http.
      | Disable - Variable is use in local only.
      mask init:
      | waijung_vdata_storage_callback('init');
      mask Help: web(fullfile(waijungdocroot,'Volatile_Data_Storage.htm'))
      mask TypeOptions storagetype: double | single | uint32 | int32 | uint16 | int16 | uint8 | int8 | string
      mask Callback storagetype: waijung_vdata_storage_callback('storagetype');
      mask Callback storagename: waijung_vdata_storage_callback('storagename');
      mask Callback initval: waijung_vdata_storage_callback('initval');
      mask Callback varname: waijung_vdata_storage_callback('varname');
      mask Callback initvalstring: waijung_vdata_storage_callback('initvalstring');
      mask TypeOptions webintegration: Disable | ReadOnly | Write/ Read | ReadOnly with KeyValuePair | Write/ Read with KeyValuePair
      mask Callback webintegration: waijung_vdata_storage_callback('webintegration');
      mask Callback weboutputformat: waijung_vdata_storage_callback('weboutputformat');
      mask TypeOptions laststoragetype: double | single | uint32 | int32 | uint16 | int16 | uint8 | int8 | string
      mask Callback sampletime: waijung_vdata_storage_callback('sampletime');
      mask Callback sampletimestr: waijung_vdata_storage_callback('sampletimestr');
      mask Callback blockid: waijung_vdata_storage_callback('blockid');
      mask Display: text(0.5, 0.5, 'Name: Line1\nType: string','ver','middle','hor','center')
  Volatile Data Storage3 : S-Function  FunctionName=waijung_vdata_storage  Parameters=storagetype,storagename,initval,varname,buffersize,initvalstring,sampletime,sampletimestr,blockid,storagetypestr  SFunctionDeploymentMode=off  EnableBusSupport=off  mask(waijung_vdata_storage){storagetype=string, storagename=Line2, initval=0, varname=VolatileDataStorage3_Line2, buffersize=64, initvalstring='', webintegration=Disable, weboutputformat='%s', webcgicallback=(void*)0, laststoragetype=string, sampletime=-1, sampletimestr=-1, blockid=VolatileDataStorage3, storagetypestr=char}
      mask prompts: storagetype "Storage Type"; storagename "Storage Name (must be a valid variable name)"; initval "Initial value (Apply at Power on Reset only)"; varname "Variable name"; buffersize "Size (bytes)"; initvalstring "Initial value (Apply at Power on Reset only)"; webintegration "Web CGI varget/varset integration"; weboutputformat "Web CGI varget output format"; webcgicallback "Web CGI varset callback"; laststoragetype "Last selected Storage Type"; sampletime "Sample time (sec)"; sampletimestr "Compiled sample time (sec) in string"; storagetypestr "Type string"
      mask help:
      | This block implements a volatile Data Storage.
      |
      | Web CGI varset/varget integratiopn:
      | Enable - In webserver application, allow remote access via http.
      | Disable - Variable is use in local only.
      mask init:
      | waijung_vdata_storage_callback('init');
      mask Help: web(fullfile(waijungdocroot,'Volatile_Data_Storage.htm'))
      mask TypeOptions storagetype: double | single | uint32 | int32 | uint16 | int16 | uint8 | int8 | string
      mask Callback storagetype: waijung_vdata_storage_callback('storagetype');
      mask Callback storagename: waijung_vdata_storage_callback('storagename');
      mask Callback initval: waijung_vdata_storage_callback('initval');
      mask Callback varname: waijung_vdata_storage_callback('varname');
      mask Callback initvalstring: waijung_vdata_storage_callback('initvalstring');
      mask TypeOptions webintegration: Disable | ReadOnly | Write/ Read | ReadOnly with KeyValuePair | Write/ Read with KeyValuePair
      mask Callback webintegration: waijung_vdata_storage_callback('webintegration');
      mask Callback weboutputformat: waijung_vdata_storage_callback('weboutputformat');
      mask TypeOptions laststoragetype: double | single | uint32 | int32 | uint16 | int16 | uint8 | int8 | string
      mask Callback sampletime: waijung_vdata_storage_callback('sampletime');
      mask Callback sampletimestr: waijung_vdata_storage_callback('sampletimestr');
      mask Callback blockid: waijung_vdata_storage_callback('blockid');
      mask Display: text(0.5, 0.5, 'Name: Line2\nType: string','ver','middle','hor','center')
  Volatile Data Storage4 : S-Function  FunctionName=waijung_vdata_storage  Parameters=storagetype,storagename,initval,varname,buffersize,initvalstring,sampletime,sampletimestr,blockid,storagetypestr  SFunctionDeploymentMode=off  EnableBusSupport=off  mask(waijung_vdata_storage){storagetype=string, storagename=Line3, initval=0, varname=VolatileDataStorage4_Line3, buffersize=64, initvalstring='', webintegration=Disable, weboutputformat='%s', webcgicallback=(void*)0, laststoragetype=string, sampletime=-1, sampletimestr=-1, blockid=VolatileDataStorage4, storagetypestr=char}
      mask prompts: storagetype "Storage Type"; storagename "Storage Name (must be a valid variable name)"; initval "Initial value (Apply at Power on Reset only)"; varname "Variable name"; buffersize "Size (bytes)"; initvalstring "Initial value (Apply at Power on Reset only)"; webintegration "Web CGI varget/varset integration"; weboutputformat "Web CGI varget output format"; webcgicallback "Web CGI varset callback"; laststoragetype "Last selected Storage Type"; sampletime "Sample time (sec)"; sampletimestr "Compiled sample time (sec) in string"; storagetypestr "Type string"
      mask help:
      | This block implements a volatile Data Storage.
      |
      | Web CGI varset/varget integratiopn:
      | Enable - In webserver application, allow remote access via http.
      | Disable - Variable is use in local only.
      mask init:
      | waijung_vdata_storage_callback('init');
      mask Help: web(fullfile(waijungdocroot,'Volatile_Data_Storage.htm'))
      mask TypeOptions storagetype: double | single | uint32 | int32 | uint16 | int16 | uint8 | int8 | string
      mask Callback storagetype: waijung_vdata_storage_callback('storagetype');
      mask Callback storagename: waijung_vdata_storage_callback('storagename');
      mask Callback initval: waijung_vdata_storage_callback('initval');
      mask Callback varname: waijung_vdata_storage_callback('varname');
      mask Callback initvalstring: waijung_vdata_storage_callback('initvalstring');
      mask TypeOptions webintegration: Disable | ReadOnly | Write/ Read | ReadOnly with KeyValuePair | Write/ Read with KeyValuePair
      mask Callback webintegration: waijung_vdata_storage_callback('webintegration');
      mask Callback weboutputformat: waijung_vdata_storage_callback('weboutputformat');
      mask TypeOptions laststoragetype: double | single | uint32 | int32 | uint16 | int16 | uint8 | int8 | string
      mask Callback sampletime: waijung_vdata_storage_callback('sampletime');
      mask Callback sampletimestr: waijung_vdata_storage_callback('sampletimestr');
      mask Callback blockid: waijung_vdata_storage_callback('blockid');
      mask Display: text(0.5, 0.5, 'Name: Line3\nType: string','ver','middle','hor','center')
  Volatile Data Storage5 : S-Function  FunctionName=waijung_vdata_storage  Parameters=storagetype,storagename,initval,varname,buffersize,initvalstring,sampletime,sampletimestr,blockid,storagetypestr  SFunctionDeploymentMode=off  EnableBusSupport=off  mask(waijung_vdata_storage){storagetype=string, storagename=Line4, initval=0, varname=VolatileDataStorage5_Line4, buffersize=64, initvalstring='', webintegration=Disable, weboutputformat='%s', webcgicallback=(void*)0, laststoragetype=string, sampletime=-1, sampletimestr=-1, blockid=VolatileDataStorage5, storagetypestr=char}
      mask prompts: storagetype "Storage Type"; storagename "Storage Name (must be a valid variable name)"; initval "Initial value (Apply at Power on Reset only)"; varname "Variable name"; buffersize "Size (bytes)"; initvalstring "Initial value (Apply at Power on Reset only)"; webintegration "Web CGI varget/varset integration"; weboutputformat "Web CGI varget output format"; webcgicallback "Web CGI varset callback"; laststoragetype "Last selected Storage Type"; sampletime "Sample time (sec)"; sampletimestr "Compiled sample time (sec) in string"; storagetypestr "Type string"
      mask help:
      | This block implements a volatile Data Storage.
      |
      | Web CGI varset/varget integratiopn:
      | Enable - In webserver application, allow remote access via http.
      | Disable - Variable is use in local only.
      mask init:
      | waijung_vdata_storage_callback('init');
      mask Help: web(fullfile(waijungdocroot,'Volatile_Data_Storage.htm'))
      mask TypeOptions storagetype: double | single | uint32 | int32 | uint16 | int16 | uint8 | int8 | string
      mask Callback storagetype: waijung_vdata_storage_callback('storagetype');
      mask Callback storagename: waijung_vdata_storage_callback('storagename');
      mask Callback initval: waijung_vdata_storage_callback('initval');
      mask Callback varname: waijung_vdata_storage_callback('varname');
      mask Callback initvalstring: waijung_vdata_storage_callback('initvalstring');
      mask TypeOptions webintegration: Disable | ReadOnly | Write/ Read | ReadOnly with KeyValuePair | Write/ Read with KeyValuePair
      mask Callback webintegration: waijung_vdata_storage_callback('webintegration');
      mask Callback weboutputformat: waijung_vdata_storage_callback('weboutputformat');
      mask TypeOptions laststoragetype: double | single | uint32 | int32 | uint16 | int16 | uint8 | int8 | string
      mask Callback sampletime: waijung_vdata_storage_callback('sampletime');
      mask Callback sampletimestr: waijung_vdata_storage_callback('sampletimestr');
      mask Callback blockid: waijung_vdata_storage_callback('blockid');
      mask Display: text(0.5, 0.5, 'Name: Line4\nType: string','ver','middle','hor','center')
  amg CLCD Setup : S-Function  FunctionName=amg_clcd  Parameters=module,configuration,inputtypearray,outputtypearray,confstr,sampletime,sampletimestr,blockid  SFunctionDeploymentMode=off  EnableBusSupport=off  mask(amg_clcd){configuration=Setup, module=1, model=amg CLCD Std, interface=4-bits, linecount=4, columncount=16, gpiotype=Push-pull, controlport=E, control_rs=7, control_rw=8, control_en=9, dataport=E, data0=12, data1=13, data2=14, data3=15, usestringbuffer=off, stringbuffer=Line2, varname=clcd_demo_4linesLCDSetupVolatileDataStorage3_Line2, inputtypearray=[0], outputtypearray=[0], confstr=["4","4","16","PP","E","7","9","8","","E","","","","","12","13","14","15","0","","0","0","0","0","1","0","0","0","0","stm32f4"], sampletime=-1, sampletimestr=-1, blockid=amgCLCDSetup}
      mask prompts: model "LCD model:"; linecount "Number of lines:"; columncount "Number of columns:"; gpiotype "GPIO Pull-Up/Down:"; controlport "GPIO control port:"; control_rs "GPIO control pin, RS:"; control_rw "GPIO control pin, RW:"; control_en "GPIO control pin, EN:"; dataport "GPIO data D[7:4] port"; data0 "GPIO data pin, D4:"; data1 "GPIO data pin, D5:"; data2 "GPIO data pin, D6:"; data3 "GPIO data pin, D7:"; usestringbuffer "Use string buffer"; stringbuffer "String buffer"; varname "Variable name"; inputtypearray "Input type array"; outputtypearray "Output type array"; confstr "Configuration string"; sampletime "Sample time (sec)"; sampletimestr "Compiled sample time (sec) in string"
      mask init:
      | amg_clcd_callback('init');
      mask Help: web(fullfile(waijungdocroot,'amg_clcd_setup.htm'), '-browser')
      mask TypeOptions configuration: Setup | Transaction
      mask Callback configuration: amg_clcd_callback('configuration');
      mask TypeOptions module: 1 | 2 | 3 | 4
      mask TypeOptions model: amg CLCD Std
      mask TypeOptions interface: 4-bits
      mask TypeOptions gpiotype: Push-pull | Open-drain
      mask TypeOptions controlport: A | B | C | D | E | F | G | H | I
      mask TypeOptions control_rs: 0 | 1 | 2 | 3 | 4 | 5 | 6 | 7 | 8 | 9 | 10 | 11 | 12 | 13 | 14 | 15
      mask TypeOptions control_rw: 0 | 1 | 2 | 3 | 4 | 5 | 6 | 7 | 8 | 9 | 10 | 11 | 12 | 13 | 14 | 15
      mask TypeOptions control_en: 0 | 1 | 2 | 3 | 4 | 5 | 6 | 7 | 8 | 9 | 10 | 11 | 12 | 13 | 14 | 15
      mask TypeOptions dataport: A | B | C | D | E | F | G | H | I
      mask TypeOptions data0: 0 | 1 | 2 | 3 | 4 | 5 | 6 | 7 | 8 | 9 | 10 | 11 | 12 | 13 | 14 | 15
      mask TypeOptions data1: 0 | 1 | 2 | 3 | 4 | 5 | 6 | 7 | 8 | 9 | 10 | 11 | 12 | 13 | 14 | 15
      mask TypeOptions data2: 0 | 1 | 2 | 3 | 4 | 5 | 6 | 7 | 8 | 9 | 10 | 11 | 12 | 13 | 14 | 15
      mask TypeOptions data3: 0 | 1 | 2 | 3 | 4 | 5 | 6 | 7 | 8 | 9 | 10 | 11 | 12 | 13 | 14 | 15
      mask Callback usestringbuffer: amg_clcd_callback('usestringbuffer');
      mask TypeOptions stringbuffer: Line3 | Line1 | Line2 | Line4
      mask Callback varname: amg_clcd_callback('varname');
      mask Callback confstr: amg_clcd_callback('confstr');
      mask Callback sampletime: amg_clcd_callback('sampletime');
      mask Callback sampletimestr: amg_clcd_callback('sampletimestr');
      mask Callback blockid: amg_clcd_callback('blockid');
      mask Display: text(0.5, 0.5, 'Module: CLCD1 (Setup)\nInterface: 4-bits\nCntrl: E7/E8/E9\nD[7:4]: E12/E13/E14/E15\nTs (sec): -1','ver','middle','hor','center');
  wires:
  Digital Input/4 -> Debounce3/1
  Digital Input/3 -> Debounce2/1
  Digital Input/2 -> Debounce1/1
  Digital Input/1 -> Debounce/1
  Digital Input1/1 -> Debounce7/1
  Debounce/1 -> Data Type Conversion7/1
  Debounce1/1 -> Data Type Conversion6/1
  Debounce2/1 -> Data Type Conversion5/1
  Debounce3/1 -> Data Type Conversion/1
  Debounce4/1 -> Data Type Conversion1/1
  Debounce5/1 -> Data Type Conversion2/1
  Debounce6/1 -> Data Type Conversion4/1
  Debounce7/1 -> Data Type Conversion3/1
  Data Type Conversion7/1 -> Gain1/1
  Data Type Conversion6/1 -> Gain/1
  Data Type Conversion5/1 -> Gain3/1
  Data Type Conversion/1 -> Gain2/1
  Data Type Conversion1/1 -> Gain4/1
  Data Type Conversion2/1 -> Gain5/1
  Data Type Conversion4/1 -> Gain6/1
  Data Type Conversion3/1 -> Gain7/1
  Gain1/1 -> Sum/1
  Gain/1 -> Sum/2
  Gain3/1 -> Sum/3
  Gain2/1 -> Sum/4
  Gain4/1 -> Sum/5
  Gain5/1 -> Sum/6
  Gain6/1 -> Sum/7
  Gain7/1 -> Sum/8
  Digital Input/5 -> Debounce5/1
  Digital Input/6 -> Debounce6/1
  Digital Input2/1 -> Debounce4/1
  Digital Input4/1 -> Debounce8/1, Debounce9/1
  Debounce8/1 -> Predator Section/Enable
  Sum/1 -> Predator Section1/1(In1)
  Debounce9/1 -> Predator Section1/Enable
  Clear/1 -> Character LCD Write/1
  Clear1/1 -> Character LCD Write/3, Character LCD Write/2
  Clear3/1 -> Character LCD Write1/2
  Clear2/1 -> Character LCD Write1/3, Character LCD Write1/1
  Mux1/1 -> Fuzzy Logic Controller/1
  Fuzzy Logic Controller/1 -> Demux/1
  Demux/1 -> Rate Transition1/1
  Demux/2 -> Rate Transition/1
  Rate Transition1/1 -> String Buffer Processing2/1
  Rate Transition/1 -> String Buffer Processing3/1
  Clear4/1 -> Character LCD Write2/1
  Clear5/1 -> Character LCD Write2/2
  Clear7/1 -> Character LCD Write3/2
  Clear6/1 -> Character LCD Write3/1
  Clear8/1 -> Character LCD Write2/3
  Clear9/1 -> Character LCD Write3/3
  Clear11/1 -> Sum2/1
  Clear10/1 -> Sum1/1
  Sum1/1 -> Mux1/1
  Sum2/1 -> Mux1/2
  Digital Input3/1 -> Debounce10/1
  Digital Input5/1 -> Debounce11/1
  Debounce11/1 -> Data Type Conversion9/1
  Debounce10/1 -> Data Type Conversion8/1
  Gain8/1 -> Sum/9
  Gain9/1 -> Sum/10
  Data Type Conversion8/1 -> Gain8/1
  Data Type Conversion9/1 -> Gain9/1
  Clear12/1 -> String Buffer Processing/1, Sum1/2
  Clear13/1 -> Sum2/2, String Buffer Processing1/1
